simulink model "rocket_plant"  (R2025b)
settings: Solver=ode4  StartTime=0.0  StopTime=200  FixedStep=0.005  RelTol=1e-3
InitFcn:
  | run(fullfile(fileparts(get_param(bdroot, 'FileName')), 'rocket_init.m'));
values from neighbouring files (symbols this model uses):
  Prk = bsim.rocket.pack(S)    [rocket_init.m]
undefined symbols (not defined in the file or in its folder): u0, x0
libraries: simulink x2
settings Model: Creator=lukascampbell  LastModifiedBy=lukascampbell
settings SFSimCC: SimCustomHeaderCode="#include \"bsim_c.h\""  SimUserIncludeDirs=/Users/lukascampbell/Documents/GitHub/6dof-uav-sim/matlab/bridge  SimUserLibraries=/Users/lukascampbell/Documents/GitHub/6dof-uav-sim/matlab/bin/libbsim_c.dylib  DefaultCustomCodeDeterministicFunctions=All

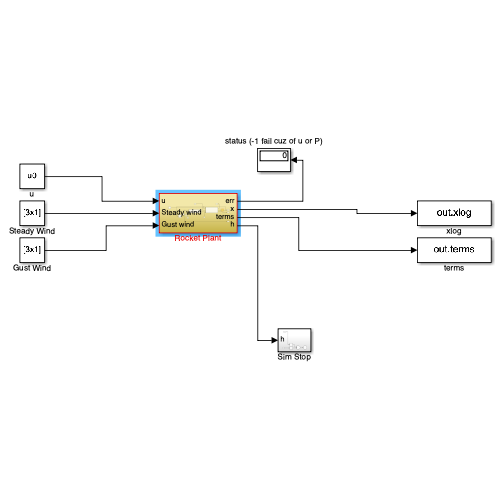
[thumbnail: Simulink's stored preview of the top-level diagram]
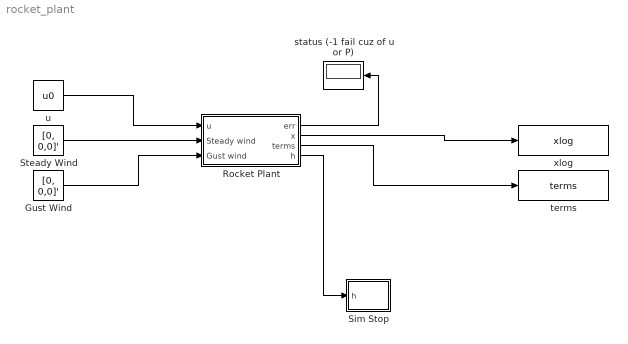
== system rocket_plant ==
  Gust Wind : Constant  Value=[0, 0,0]'
  Rocket Plant : Subsystem
  Sim Stop : Subsystem
  Steady Wind : Constant  Value=[0, 0,0]'
  status (-1 fail cuz of u or P) : Display
  terms : ToWorkspace  VariableName=terms  SaveFormat=Timeseries  SampleTime=-1
  u : Constant  Value=u0
  xlog : ToWorkspace  VariableName=xlog  SaveFormat=Timeseries  SampleTime=-1
  wires:
  Rocket Plant/1(err) -> status (-1 fail cuz of u or P)/1
  Steady Wind/1 -> Rocket Plant/2(Steady wind)
  Gust Wind/1 -> Rocket Plant/3(Gust wind)
  Rocket Plant/2(x) -> xlog/1
  Rocket Plant/3(terms) -> terms/1
  u/1 -> Rocket Plant/1(u)
  Rocket Plant/4(h) -> Sim Stop/1(h)

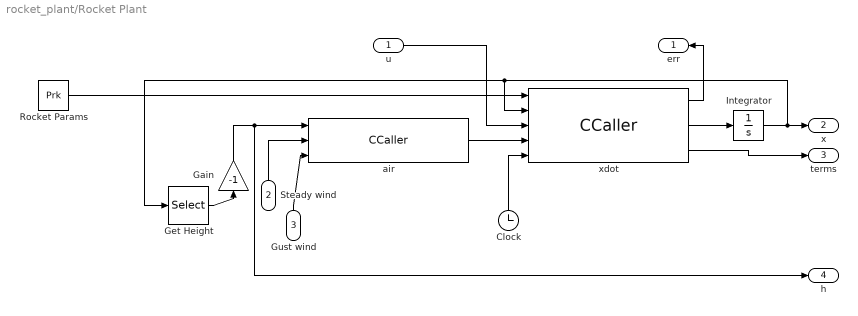
== system rocket_plant/Rocket Plant ==
  u : Inport
  Steady wind : Inport  Port=2
  Gust wind : Inport  Port=3
  Clock : Clock
  Gain : Gain  Gain=-1
  Get Height : Selector  InputPortWidth=14  IndexOptions=Index vector (dialog)  Indices=3  OutputSizes=1
  Integrator : Integrator  InitialCondition=x0
  Rocket Params : Constant  Value=Prk
  air : CCaller  FunctionName=bsim_isa_rocket_air  PortSpecificationStruct="%)30     .    & <   8    (     @         %    \"     0    !     0         %  0 \"0    $    _    07)G3F%M90  4&]R=$YA;64 4V-O<&4     26YD97@     5'EP90      4VEZ90      27-';&]B86P   X    P    !@    @    $          4    (     0    $    !         !   0!H    #@   #     &    \"     0         !0    @    !     0    $         $  ! &@    .    .     8    (    !          %    \"     $    %     0         0   ...(+2058 chars)"
  xdot : CCaller  FunctionName=bsim_rocket_xdot  PortSpecificationStruct="%)30     .    Z!    8    (     @         %    \"     H    !     0         %  0 \"0    $    _    07)G3F%M90  4&]R=$YA;64 4V-O<&4     26YD97@     5'EP90      4VEZ90      27-';&]B86P   X    P    !@    @    $          4    (     0    ,    !         !   P!O=70 #@   #     &    \"     0         !0    @    !     P    $         $  # &]U=  .    .     8    (    !          %    \"     $    &     0         0   ...(+5457 chars)"
  err : Outport
  x : Outport  Port=2
  terms : Outport  Port=3
  h : Outport  Port=4
  wires:
  Get Height/1 -> Gain/1
  air/1 -> xdot/4
  Gust wind/1 -> air/3
  Integrator/1 -> x/1, xdot/2, Get Height/1
  xdot/2 -> Integrator/1
  Steady wind/1 -> air/2
  u/1 -> xdot/3
  xdot/1 -> err/1
  Rocket Params/1 -> xdot/1
  Clock/1 -> xdot/5
  Gain/1 -> h/1, air/1
  xdot/3 -> terms/1

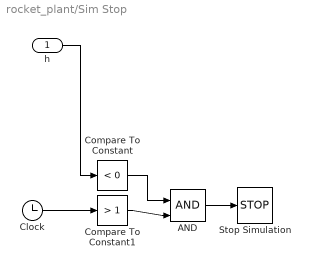
== system rocket_plant/Sim Stop ==
  h : Inport
  AND : Logic  IconShape=distinctive  AllPortsSameDT=off  OutDataTypeStr=boolean
  Clock : Clock
  Compare To Constant : simulink/Logic and Bit Operations/Compare To Constant  relop=<  const=0  OutDataTypeStr=boolean
  Compare To Constant1 : simulink/Logic and Bit Operations/Compare To Constant  relop=>  const=1  OutDataTypeStr=boolean
  Stop Simulation : Stop
  wires:
  AND/1 -> Stop Simulation/1
  Compare To Constant/1 -> AND/1
  h/1 -> Compare To Constant/1
  Compare To Constant1/1 -> AND/2
  Clock/1 -> Compare To Constant1/1
